simulink model "Exp3"  (R2025b)
settings: Solver=VariableStepAuto  StartTime=0.0  StopTime=10.0  RelTol=1e-3
libraries: hdlsllib x4
settings Model: Creator=SUBHASH  LastModifiedBy=SUBHASH

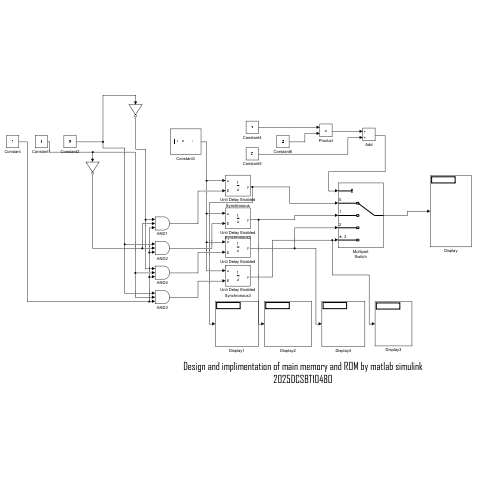
[thumbnail: Simulink's stored preview of the top-level diagram]
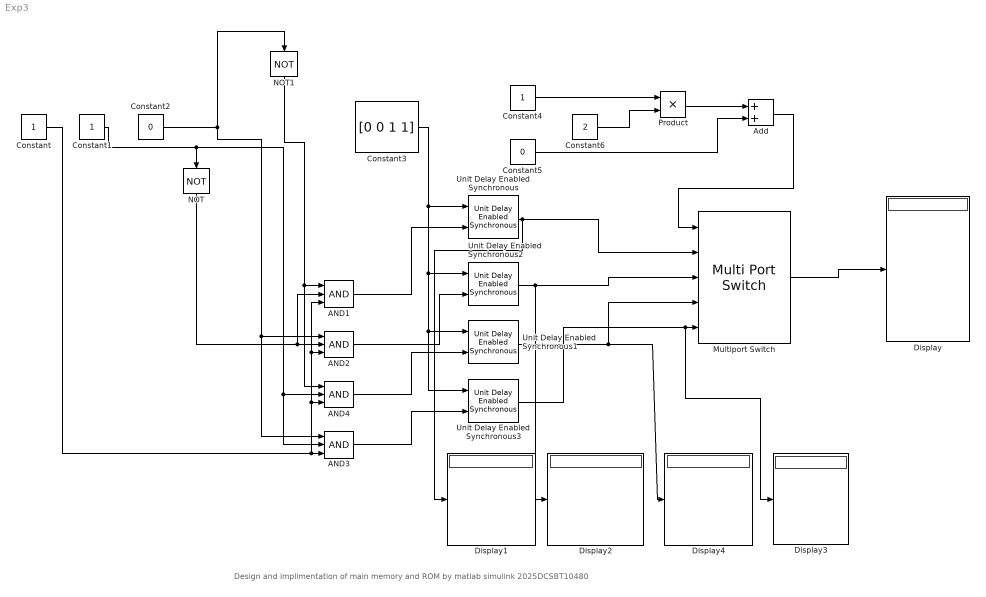
== system Exp3 ==
  note: Design and implimentation of main memory and ROM by matlab simulink
      | 2025DCSBT10480
  AND{1..4} (4 alike) : Logic  Inputs=3  IconShape=distinctive  AllPortsSameDT=off  OutDataTypeStr=boolean
  Add : Sum
  Constant : Constant
  Constant1 : Constant
  Constant2 : Constant  Value=0
  Constant3 : Constant  Value=[0 0 1 1]
  Constant4 : Constant
  Constant5 : Constant  Value=0
  Constant6 : Constant  Value=2
  Display{,1..4} (5 alike) : Display
  Multiport Switch : MultiPortSwitch  DataPortOrder=Zero-based contiguous  Inputs=4  zeroidx=on  SaturateOnIntegerOverflow=off  InputSameDT=off
  NOT : Logic  Operator=NOT  IconShape=distinctive  AllPortsSameDT=off  OutDataTypeStr=boolean
  NOT1 : Logic  Operator=NOT  IconShape=distinctive  AllPortsSameDT=off  OutDataTypeStr=boolean
  Product : Product
  Unit Delay Enabled Synchronous{,1..3} (4 alike) : hdlsllib/Discrete/Unit Delay Enabled Synchronous  InitialCondition=0.0  SampleTime=-1
  wires:
  Constant1/1 -> AND4/2, AND3/2, NOT/1
  Constant2/1 -> NOT1/1, AND2/1, AND3/1
  Constant/1 -> AND1/3, AND2/3, AND4/3, AND3/3
  NOT/1 -> AND2/2, AND1/2
  NOT1/1 -> AND1/1, AND4/1
  Constant4/1 -> Product/1
  Constant6/1 -> Product/2
  Constant5/1 -> Add/2
  Product/1 -> Add/1
  Add/1 -> Multiport Switch/1
  Multiport Switch/1 -> Display/1
  AND1/1 -> Unit Delay Enabled Synchronous/2
  AND2/1 -> Unit Delay Enabled Synchronous2/2
  AND4/1 -> Unit Delay Enabled Synchronous1/2
  AND3/1 -> Unit Delay Enabled Synchronous3/2
  Constant3/1 -> Unit Delay Enabled Synchronous/1, Unit Delay Enabled Synchronous2/1, Unit Delay Enabled Synchronous1/1, Unit Delay Enabled Synchronous3/1
  Unit Delay Enabled Synchronous/1 -> Display1/1, Multiport Switch/2
  Unit Delay Enabled Synchronous2/1 -> Display2/1, Multiport Switch/3
  Unit Delay Enabled Synchronous1/1 -> Display4/1, Multiport Switch/4
  Unit Delay Enabled Synchronous3/1 -> Display3/1, Multiport Switch/5
